simulink model "q_hover"  (R2024a)
settings: Solver=ode1  StartTime=0.0  StopTime=inf  FixedStep=0.002  RelTol=1e-3  EnableMultiTasking=on
values from neighbouring files (symbols this model uses):
  CMD_RATE_LIMIT = 60 * pi/180    (= 1.0471975512)    [setup_lab_hover.m]
  INT_JOYSTICK_SAT_LOWER = -10    [setup_lab_hover.m]
  INT_JOYSTICK_SAT_UPPER = 10    [setup_lab_hover.m]
  JOYSTICK_X_DZ = 0.25    [setup_lab_hover.m]
  JOYSTICK_Y_DZ = 0.25    [setup_lab_hover.m]
  K = lqr( A, B, Q, R )    [setup_lab_hover.m]
  K_AMP = 3    [setup_lab_hover.m]
  K_EC_P = 2 * pi / ( 8 * 1024 )    (= 0.000766990393943)    [config_hover.m]
  K_EC_R = 2 * pi / ( 8 * 1024 )    (= 0.000766990393943)    [config_hover.m]
  K_EC_Y = -2 * pi / ( 8 * 1024 )    (= -0.000766990393943)    [config_hover.m]
  K_JOYSTICK_X = -25    [setup_lab_hover.m]
  K_JOYSTICK_Y = 25    [setup_lab_hover.m]
  V_bias = 2.0    (= 2)    [setup_lab_hover.m]
  VMAX_AMP = 24    [setup_lab_hover.m]
  wcf = 2 * pi * 20    (= 125.663706144)    [setup_lab_hover.m]
  zetaf = 0.8    [setup_lab_hover.m]
undefined symbols (not defined in the file or in its folder): HIL, qc_get_step_size
libraries: simulink_extras x6, quarc_library x4
settings Model: SimulationMode=external  ExtModeTrigDuration=10000  Creator=hpineros  LastModifiedBy=user
settings SolverCC: AlgebraicLoopSolver=TrustRegion  PositivePriorityOrder=on
settings DataIOCC: LimitDataPoints=on  SaveFormat=Array  SignalLoggingSaveFormat=ModelDataLogs  ReturnWorkspaceOutputs=off
settings OptimizationCC: ExpressionDepthLimit=2147483647  InitFltsAndDblsToZero=on
settings DebuggingCC: SaveWithParameterizedLinksMsg=none  UnderspecifiedInitializationDetection=Classic  MergeDetectMultiDrivingBlocksExec=none  SolverPrmCheckMsg=warning  FcnCallInpInsideContextMsg=warning  UnconnectedInputMsg=warning  UnconnectedOutputMsg=warning  UnconnectedLineMsg=warning  StateNameClashWarn=warning  SFUnexpectedBacktrackingDiag=warning  SFNoUnconditionalDefaultTransitionDiag=warning  SFExecutionAtInitializationDiag=none  ArithmeticOperatorsInVariantConditions=warning
settings ModelReferenceCC: PropagateSignalLabelsOutOfModel=off
settings SFSimCC: SimUseLocalCustomCode=off  CustomCodeUndefinedFunction=UseInterfaceOnly
settings RTWCC: Description=QUARC Win64 Target Using Toolchain  SystemTargetFile=quarc_win64.tlc  TemplateMakefile=quarc_default_tmf  RTWUseLocalCustomCode=off  Toolchain=QUARC win64 | nmake (64-bit Windows)  BuildConfiguration=Faster Runs  GPUComputeCapability=3.5
settings CodeAppCC: StateflowObjectComments=on
settings STFCustomTargetCC: TargetLangStandard=C89/C90 (ANSI)  ConcurrentExecutionCompliant=on  SystemTargetFile=quarc_win64.tlc
settings GRTTargetCC: TargetLangStandard=C89/C90 (ANSI)  ParMdlRefBuildCompliant=off  CompOptLevelCompliant=off  CombineOutputUpdateFcns=off  MatFileLogging=off  CPPClassGenCompliant=off  GRTInterface=on  ExtMode=on  ExtModeMexFile=quarc_comm
settings ConfigComp: CovMetricSettings=dw  CovSaveCumulativeToWorkspaceVar=on  CovSaveSingleToWorkspaceVar=on  CovExternalEMLEnable=off

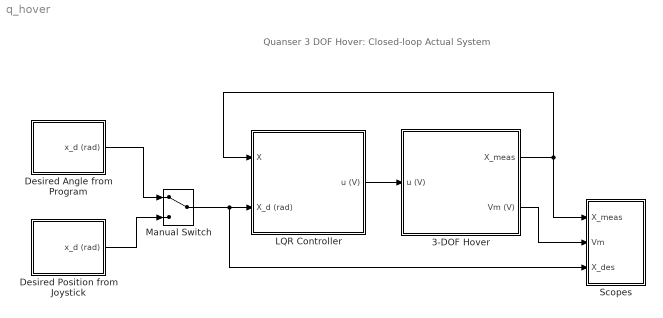
== system q_hover ==
  note: Quanser 3 DOF Hover:
      | Closed-loop Actual System
  3-DOF Hover : Subsystem
  Desired Angle from Program : Subsystem
  Desired Position from Joystick : Subsystem
  LQR Controller : Subsystem
  Manual Switch : ManualSwitch
  Scopes : Subsystem
  wires:
  3-DOF Hover/1(X_meas) -> LQR Controller/1(X), Scopes/1(X_meas)
  3-DOF Hover/2(Vm (V)) -> Scopes/2(Vm)
  Desired Angle from Program/1(x_d (rad)) -> Manual Switch/1
  Desired Position from Joystick/1(x_d (rad)) -> Manual Switch/2
  Manual Switch/1 -> Scopes/3(X_des), LQR Controller/2(X_d (rad))
  LQR Controller/1(u (V)) -> 3-DOF Hover/1(u (V))

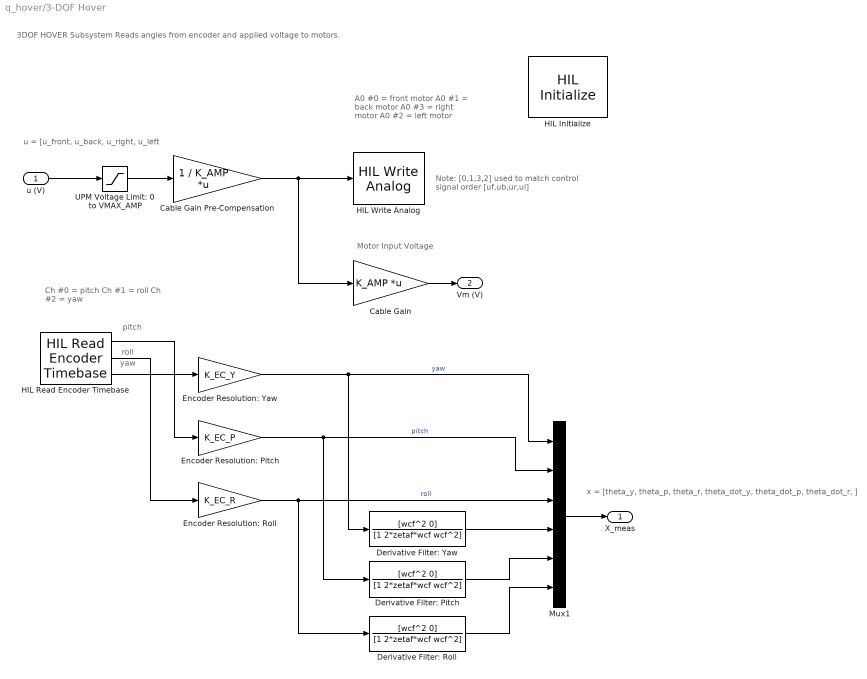
== system q_hover/3-DOF Hover ==
  note: Note: [0,1,3,2] used to match
      | control signal order [uf,ub,ur,ul]
  note: roll
  note: pitch
  note: yaw
  note: Motor Input Voltage
  note: x = [theta_y, theta_p, theta_r, theta_dot_y, theta_dot_p, theta_dot_r, ]
  note: A0 #0 = front motor
      | A0 #1 = back motor
      | A0 #3 = right motor
      | A0 #2 = left motor
  note: u = [u_front, u_back, u_right, u_left
  note: 3DOF HOVER Subsystem
      | Reads angles from encoder and applied voltage to motors.
  note: Ch #0 = pitch
      | Ch #1 = roll
      | Ch #2 = yaw
  u (V) : Inport
  Cable Gain : Gain  Gain=K_AMP  Multiplication=Matrix(K*u)  SaturateOnIntegerOverflow=on  OutDataTypeStr=Inherit: Same as input  ParamDataTypeStr=Inherit: Same as input
  Cable Gain Pre-Compensation : Gain  Gain=1 / K_AMP  Multiplication=Matrix(K*u)  SaturateOnIntegerOverflow=on  OutDataTypeStr=Inherit: Same as input  ParamDataTypeStr=Inherit: Same as input
  Derivative Filter: Pitch : TransferFcn  Numerator=[wcf^2 0]  Denominator=[1 2*zetaf*wcf wcf^2]
  Derivative Filter: Roll : TransferFcn  Numerator=[wcf^2 0]  Denominator=[1 2*zetaf*wcf wcf^2]
  Derivative Filter: Yaw : TransferFcn  Numerator=[wcf^2 0]  Denominator=[1 2*zetaf*wcf wcf^2]
  Encoder Resolution: Pitch : Gain  Gain=K_EC_P
  "Encoder Resolution: Roll " : Gain  Gain=K_EC_R
  Encoder Resolution: Yaw : Gain  Gain=K_EC_Y
  HIL Initialize : quarc_library/Data Acquisition/Generic/Configuration/HIL Initialize  object_name=HIL-1  board_type=q8_usb  board_number=0  board_options=update_rate=normal  exclusive=off  active=on  hardware_clocks=[0:2]  clock_modes=[]  initial_clock_frequencies=[]  set_clock_params_at_start=off  set_clock_params_at_switch_in=off  set_clock_frequencies_at_start=off  set_clock_frequencies_at_switch_in=off  analog_input_channels=[0:7]  analog_input_configurations=[]  analog_input_maximums=10  analog_input_minimums=-10  set_analog_input_params_at_start=on  set_analog_input_params_at_switch_in=off  analog_output_channels=[0:7]  analog_output_maximums=10  analog_output_minimums=-10  initial_analog_outputs=[0]  final_analog_outputs=[0]  watchdog_analog_outputs=0  set_analog_output_params_at_start=on  set_analog_output_params_at_switch_in=off  set_analog_outputs_at_start=on  set_analog_outputs_at_switch_in=off  set_analog_outputs_at_terminate=on  set_analog_outputs_at_switch_out=off  set_analog_outputs_on_watchdog=off  digital_input_channels=[]  digital_output_channels=[0:3]  digital_output_configuration=[]  initial_digital_outputs=[0]  final_digital_outputs=[0]  watchdog_digital_outputs=[0]  set_digital_output_params_at_start=off  set_digital_output_params_at_switch_in=off  set_digital_outputs_at_start=on  set_digital_outputs_at_switch_in=off  set_digital_outputs_at_terminate=on  set_digital_outputs_at_switch_out=off  set_digital_outputs_on_watchdog=off  encoder_channels=[0:7]  quadrature=[4]  encoder_filter_frequency=[]  initial_encoder_counts=[0]  set_encoder_params_at_start=on  set_encoder_params_at_switch_in=off  set_encoder_counts_at_start=on  set_encoder_counts_at_switch_in=off  pwm_channels=[0:7]  pwm_modes=0  pwm_frequency=99.532799999999995e6/4095  pwm_configuration=[0]  pwm_alignment=[0]  pwm_polarity=[1]  pwm_leading_deadband=[0]  pwm_trailing_deadband=[0]  initial_pwm_outputs=[0]  final_pwm_outputs=[0]  watchdog_pwm_outputs=[0]  set_pwm_params_at_start=on  set_pwm_params_at_switch_in=off  set_pwm_outputs_at_start=on  set_pwm_outputs_at_switch_in=off  set_pwm_outputs_at_terminate=on  set_pwm_outputs_at_switch_out=off  set_pwm_outputs_on_watchdog=off  other_output_channels=[]  initial_other_outputs=[]  final_other_outputs=[]  watchdog_other_outputs=[]  set_other_outputs_at_start=off  set_other_outputs_at_switch_in=off  set_other_outputs_at_terminate=off  set_other_outputs_at_switch_out=off  set_other_outputs_on_watchdog=off
  HIL Read Encoder Timebase : quarc_library/Data Acquisition/Generic/Timebases/HIL Read Encoder Timebase  object_name=HIL-1  clock=0  channels=[0:2]  active=on  vector_output=off  data_type_mode=Inherit via back propagation  data_type=double  overflow_mode=Error on overflow  samples_in_buffer=max(ceil(1/qc_get_step_size), 1)
  HIL Write Analog : quarc_library/Data Acquisition/Generic/Immediate I//O/HIL Write Analog  object_name=HIL-1  channels=[0,1,3,2]  sample_time=-1  active=off  vector_input=on
  Mux1 : Mux  Inputs=6
  UPM Voltage Limit: 0 to VMAX_AMP : Saturate  UpperLimit=VMAX_AMP  LowerLimit=0
  X_meas : Outport
  Vm (V) : Outport  Port=2
  wires:
  Cable Gain Pre-Compensation/1 -> Cable Gain/1, HIL Write Analog/1
  HIL Read Encoder Timebase/3 -> Encoder Resolution: Yaw/1
  HIL Read Encoder Timebase/1 -> Encoder Resolution: Pitch/1
  HIL Read Encoder Timebase/2 -> "Encoder Resolution: Roll "/1
  Mux1/1 -> X_meas/1
  UPM Voltage Limit: 0 to VMAX_AMP/1 -> Cable Gain Pre-Compensation/1
  Cable Gain/1 -> Vm (V)/1
  u (V)/1 -> UPM Voltage Limit: 0 to VMAX_AMP/1
  Encoder Resolution: Yaw/1 -> Mux1/1, Derivative Filter: Yaw/1  "yaw"
  Encoder Resolution: Pitch/1 -> Mux1/2, Derivative Filter: Pitch/1  "pitch"
  "Encoder Resolution: Roll "/1 -> Mux1/3, Derivative Filter: Roll/1  "roll"
  Derivative Filter: Yaw/1 -> Mux1/4
  Derivative Filter: Pitch/1 -> Mux1/5
  Derivative Filter: Roll/1 -> Mux1/6

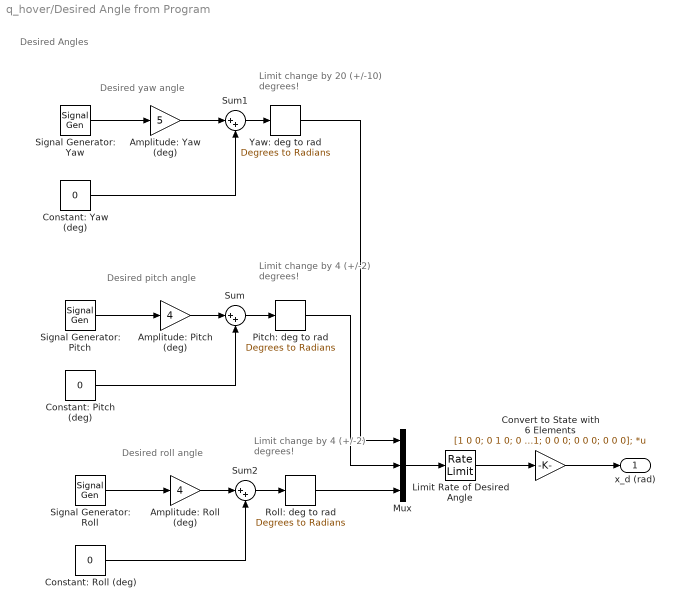
== system q_hover/Desired Angle from Program ==
  note: Desired Angles
  note: Limit change by
      | 4 (+/-2) degrees!
  note: Limit change by
      | 20 (+/-10) degrees!
  note: Limit change by
      | 4 (+/-2) degrees!
  note: Desired roll angle
  note: Desired pitch angle
  note: Desired yaw angle
  Amplitude: Pitch (deg) : Gain  Gain=4
  Amplitude: Roll (deg) : Gain  Gain=4
  Amplitude: Yaw (deg) : Gain  Gain=5
  Constant: Pitch (deg) : Constant  Value=0
  Constant: Roll (deg) : Constant  Value=0
  Constant: Yaw (deg) : Constant  Value=0
  Convert to State with 6 Elements : Gain  Gain=[1 0 0; 0 1 0; 0 0 1; 0 0 0; 0 0 0; 0 0 0];  Multiplication=Matrix(K*u)
  Limit Rate of Desired Angle : RateLimiter  RisingSlewLimit=CMD_RATE_LIMIT  FallingSlewLimit=-CMD_RATE_LIMIT
  Mux : Mux  Inputs=3
  Pitch: deg to rad : simulink_extras/Transformations/Degrees to Radians
  Roll: deg to rad : simulink_extras/Transformations/Degrees to Radians
  Signal Generator: Pitch : SignalGenerator  WaveForm=square  Frequency=0.1
  Signal Generator: Roll : SignalGenerator  WaveForm=square  Frequency=0.08
  Signal Generator: Yaw : SignalGenerator  WaveForm=square  Frequency=0.04
  Sum : Sum  Inputs=|++
  Sum1 : Sum  Inputs=|++
  Sum2 : Sum  Inputs=|++
  Yaw: deg to rad : simulink_extras/Transformations/Degrees to Radians
  x_d (rad) : Outport
  wires:
  Convert to State with 6 Elements/1 -> x_d (rad)/1
  Limit Rate of Desired Angle/1 -> Convert to State with 6 Elements/1
  Roll: deg to rad/1 -> Mux/3
  Pitch: deg to rad/1 -> Mux/2
  Yaw: deg to rad/1 -> Mux/1
  Sum2/1 -> Roll: deg to rad/1
  Signal Generator: Roll/1 -> Amplitude: Roll (deg)/1
  Amplitude: Roll (deg)/1 -> Sum2/1
  Constant: Roll (deg)/1 -> Sum2/2
  Sum/1 -> Pitch: deg to rad/1
  Signal Generator: Pitch/1 -> Amplitude: Pitch (deg)/1
  Amplitude: Pitch (deg)/1 -> Sum/1
  Constant: Pitch (deg)/1 -> Sum/2
  Sum1/1 -> Yaw: deg to rad/1
  Signal Generator: Yaw/1 -> Amplitude: Yaw (deg)/1
  Amplitude: Yaw (deg)/1 -> Sum1/1
  Constant: Yaw (deg)/1 -> Sum1/2
  Mux/1 -> Limit Rate of Desired Angle/1

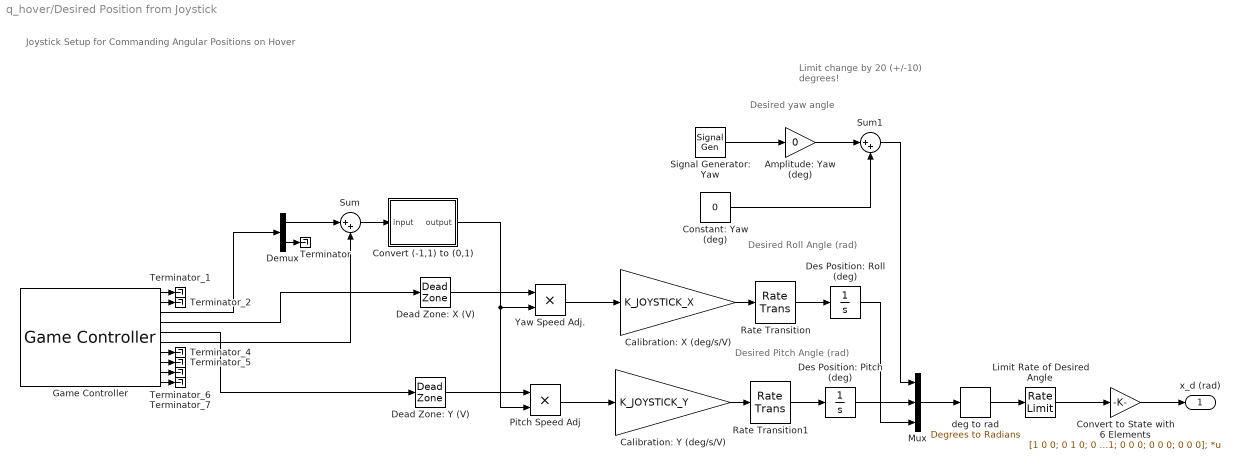
== system q_hover/Desired Position from Joystick ==
  note: Limit change by
      | 20 (+/-10) degrees!
  note: Desired yaw angle
  note: Desired Roll Angle (rad)
  note: Desired Pitch Angle (rad)
  note: Joystick Setup for Commanding Angular Positions on Hover
  Amplitude: Yaw (deg) : Gain  Gain=0
  Calibration: X (deg/s/V) : Gain  Gain=K_JOYSTICK_X
  Calibration: Y (deg/s/V) : Gain  Gain=K_JOYSTICK_Y
  Constant: Yaw (deg) : Constant  Value=0
  Convert (-1,1) to (0,1) : Subsystem
  Convert to State with 6 Elements : Gain  Gain=[1 0 0; 0 1 0; 0 0 1; 0 0 0; 0 0 0; 0 0 0];  Multiplication=Matrix(K*u)
  Dead Zone: X (V) : DeadZone  LowerValue=-JOYSTICK_X_DZ  UpperValue=JOYSTICK_X_DZ
  Dead Zone: Y (V) : DeadZone  LowerValue=-JOYSTICK_Y_DZ  UpperValue=JOYSTICK_Y_DZ
  Demux : Demux  Outputs=2
  Des Position: Pitch (deg) : Integrator  LimitOutput=on  UpperSaturationLimit=INT_JOYSTICK_SAT_UPPER  LowerSaturationLimit=INT_JOYSTICK_SAT_LOWER
  Des Position: Roll (deg) : Integrator  LimitOutput=on  UpperSaturationLimit=INT_JOYSTICK_SAT_UPPER  LowerSaturationLimit=INT_JOYSTICK_SAT_LOWER
  Game Controller : quarc_library/Devices/Peripherals/Target/Game Controller  controller=1  buffer_size=12  deadzone=[]  saturation=[]  sample_time=max(qc_get_step_size, 0.01)  auto_center=off  enabled=on
      settings: SourceProductName=QUARC Targets
  Limit Rate of Desired Angle : RateLimiter  RisingSlewLimit=CMD_RATE_LIMIT  FallingSlewLimit=-CMD_RATE_LIMIT
  Mux : Mux  Inputs=3
  Pitch Speed Adj : Product  RndMeth=Zero
  Rate Transition : RateTransition
  Rate Transition1 : RateTransition
  Signal Generator: Yaw : SignalGenerator  WaveForm=square  Frequency=0.04
  Sum : Sum  Inputs=|++
  Sum1 : Sum  Inputs=|++
  Terminator : Terminator
  Terminator_{1..2,4..7} (6 alike) : Terminator
  Yaw Speed Adj. : Product  RndMeth=Zero
  deg to rad : simulink_extras/Transformations/Degrees to Radians
  x_d (rad) : Outport
  wires:
  Sum1/1 -> Mux/1
  Signal Generator: Yaw/1 -> Amplitude: Yaw (deg)/1
  Amplitude: Yaw (deg)/1 -> Sum1/1
  Constant: Yaw (deg)/1 -> Sum1/2
  Limit Rate of Desired Angle/1 -> Convert to State with 6 Elements/1
  Mux/1 -> deg to rad/1
  deg to rad/1 -> Limit Rate of Desired Angle/1
  Convert to State with 6 Elements/1 -> x_d (rad)/1
  Calibration: X (deg/s/V)/1 -> Rate Transition/1
  Dead Zone: X (V)/1 -> Yaw Speed Adj./1
  Dead Zone: Y (V)/1 -> Pitch Speed Adj/1
  Yaw Speed Adj./1 -> Calibration: X (deg/s/V)/1
  Pitch Speed Adj/1 -> Calibration: Y (deg/s/V)/1
  Calibration: Y (deg/s/V)/1 -> Rate Transition1/1
  Convert (-1,1) to (0,1)/1(output) -> Yaw Speed Adj./2, Pitch Speed Adj/2
  Rate Transition/1 -> Des Position: Roll (deg)/1
  Des Position: Roll (deg)/1 -> Mux/3
  Des Position: Pitch (deg)/1 -> Mux/2
  Rate Transition1/1 -> Des Position: Pitch (deg)/1
  Game Controller/4 -> Dead Zone: X (V)/1
  Game Controller/5 -> Dead Zone: Y (V)/1
  Game Controller/1 -> Terminator_1/1
  Game Controller/2 -> Terminator_2/1
  Game Controller/7 -> Terminator_4/1
  Game Controller/8 -> Terminator_5/1
  Game Controller/9 -> Terminator_6/1
  Game Controller/10 -> Terminator_7/1
  Sum/1 -> Convert (-1,1) to (0,1)/1(input)
  Game Controller/6 -> Sum/2
  Demux/1 -> Sum/1
  Game Controller/3 -> Demux/1
  Demux/2 -> Terminator/1

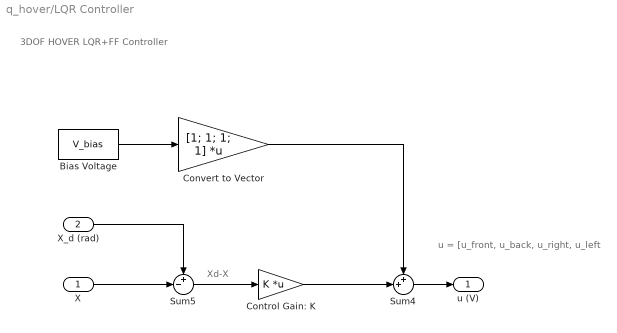
== system q_hover/LQR Controller ==
  note: u = [u_front, u_back, u_right, u_left
  note: Xd-X
  note: 3DOF HOVER LQR+FF Controller
  X : Inport
  X_d (rad) : Inport  Port=2
  Bias Voltage : Constant  Value=V_bias
  Control Gain: K : Gain  Gain=K  Multiplication=Matrix(K*u)
  Convert to Vector : Gain  Gain=[1; 1; 1; 1]  Multiplication=Matrix(K*u)
  Sum4 : Sum  Inputs=++|
  Sum5 : Sum  Inputs=+-|
  u (V) : Outport
  wires:
  Sum5/1 -> Control Gain: K/1
  X/1 -> Sum5/2
  X_d (rad)/1 -> Sum5/1
  Convert to Vector/1 -> Sum4/1
  Control Gain: K/1 -> Sum4/2
  Bias Voltage/1 -> Convert to Vector/1
  Sum4/1 -> u (V)/1

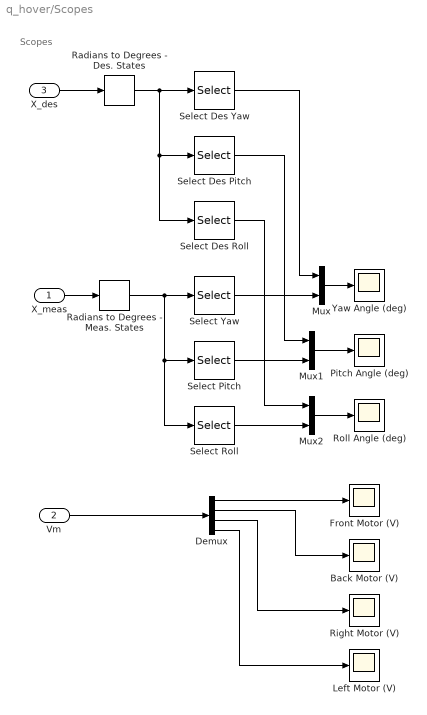
== system q_hover/Scopes ==
  note: Scopes
  X_meas : Inport
  Vm : Inport  Port=2
  X_des : Inport  Port=3
  Back Motor (V) : Scope
  Demux : Demux
  Front Motor (V) : Scope
  Left Motor (V) : Scope
  Mux : Mux  Inputs=2
  Mux1 : Mux  Inputs=2
  Mux2 : Mux  Inputs=2
  Pitch Angle (deg) : Scope
  Radians to Degrees - Des. States : simulink_extras/Transformations/Radians to Degrees
  Radians to Degrees - Meas. States : simulink_extras/Transformations/Radians to Degrees
  Right Motor (V) : Scope
  Roll Angle (deg) : Scope
  Select Des Pitch : Selector  InputPortWidth=6  IndexOptions=Index vector (dialog)  Indices=2  OutputSizes=1
  Select Des Roll : Selector  InputPortWidth=6  IndexOptions=Index vector (dialog)  Indices=3  OutputSizes=1
  Select Des Yaw : Selector  InputPortWidth=6  IndexOptions=Index vector (dialog)  Indices=1  OutputSizes=1
  Select Pitch : Selector  InputPortWidth=6  IndexOptions=Index vector (dialog)  Indices=2  OutputSizes=1
  Select Roll : Selector  InputPortWidth=6  IndexOptions=Index vector (dialog)  Indices=3  OutputSizes=1
  Select Yaw : Selector  InputPortWidth=6  IndexOptions=Index vector (dialog)  Indices=1  OutputSizes=1
  Yaw Angle (deg) : Scope
  wires:
  Demux/4 -> Left Motor (V)/1
  Demux/3 -> Right Motor (V)/1
  Demux/2 -> Back Motor (V)/1
  Demux/1 -> Front Motor (V)/1
  Vm/1 -> Demux/1
  X_des/1 -> Radians to Degrees - Des. States/1
  X_meas/1 -> Radians to Degrees - Meas. States/1
  Mux/1 -> Yaw Angle (deg)/1
  Mux1/1 -> Pitch Angle (deg)/1
  Radians to Degrees - Meas. States/1 -> Select Yaw/1, Select Pitch/1, Select Roll/1
  Mux2/1 -> Roll Angle (deg)/1
  Select Yaw/1 -> Mux/2
  Select Pitch/1 -> Mux1/2
  Select Roll/1 -> Mux2/2
  Radians to Degrees - Des. States/1 -> Select Des Yaw/1, Select Des Pitch/1, Select Des Roll/1
  Select Des Yaw/1 -> Mux/1
  Select Des Pitch/1 -> Mux1/1
  Select Des Roll/1 -> Mux2/1

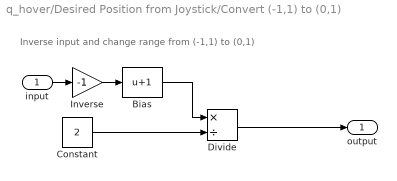
== system q_hover/Desired Position from Joystick/Convert (-1,1) to (0,1) ==
  note: Inverse input and change range from (-1,1) to (0,1)
  input : Inport
  Bias : Bias  Bias=1  SaturateOnIntegerOverflow=off
  Constant : Constant  Value=2
  Divide : Product  Inputs=*/
  Inverse : Gain  Gain=-1
  output : Outport
  wires:
  Bias/1 -> Divide/1
  input/1 -> Inverse/1
  Divide/1 -> output/1
  Inverse/1 -> Bias/1
  Constant/1 -> Divide/2
